simulink model "sm_wheel_loader_steer"  (R2025a)
settings: Solver=ode23t  StartTime=0.0  StopTime=70  RelTol=1e-3  AbsTol=1e-3
libraries: fl_lib x13, sm_wheel_loader_lib x6, sm_lib x3, SimscapeFluids_lib x1, nesl_utility x1
CloseFcn:
  | clear simlog_sm_wheel_loader_steering
  | clear logsout_sm_wheel_loader_steering
Description:
  | Copyright 2024-2025 The MathWorks, Inc.
settings Model: Creator=smiller  LastModifiedBy=smiller
settings SolverCC: AutoScaleAbsTol=off  AlgebraicLoopSolver=TrustRegion  MaxZcPerStep=1.0
settings DataIOCC: MaxDataPoints=10000  ReturnWorkspaceOutputs=off  SignalLoggingName=logsout_sm_wheel_loader_steer
settings DebuggingCC: UnconnectedInputMsg=warning  UnconnectedOutputMsg=warning  UnconnectedLineMsg=warning  SymbolicDimsDataTypeCodeGenerationDiagnostic=none
settings ModelReferenceCC: EnableRefExpFcnMdlSchedulingChecks=on
settings SFSimCC: CustomCodeUndefinedFunction=UseInterfaceOnly
settings RTWCC: GPUComputeCapability=3.5  DLArmComputeVersion=19.05
settings SimscapeCC: SimscapeLogType=all  SimscapeLogSimulationStatistics=on  SimscapeLogName=simlog_sm_wheel_loader_steer  SimscapeLogLimitData=off  SimscapeLogDataHistory=10000.0
settings DiagnosticsConfigSet: SimMechanicsUnconnectedFramePorts=none  SimMechanicsConflictingReferenceFrames=none
settings ExplorerConfigSet: InternalSimMechanicsExplorerSettings="<ExplorerConfiguration><canonicalview>default</canonicalview><AnimationSetting><BasePlaybackSpeed>1.0</BasePlaybackSpeed><PlaybackSpeedFactor>4.0</PlaybackSpeedFactor></AnimationSetting><TilePanel><TileInfo><Tiles Columns=\"2\" Count=\"2\" Rows=\"1\"><Column Weight=\"0.6653\"/><Column Weight=\"0.3347\"/><Row Weight=\"1\"/><Tile Height=\"1\" Width=\"1\" X=\"0\" Y=\"0\"/><Tile Height=\"1\" Width=\"1\" X=\"1\" Y=\"0\"/></Tiles></TileInfo><SceneInfo><SceneViewer><BGColor><R>1</R><G>1</G><B>1</B></BGColor><Camera><DoPerspective>off</DoPerspective><Position><X>-1.6762096275510312</X><Y>0.728440342877136993</Y><Z>1.10654866732435075</Z></Position><Center><X>0.0428012803943581543</X><Y>-0.54445752799199687</Y><Z>0.718090657281730271</Z></Center><Up><X>0.119453996973749921</X><Y>-0.138700664007791685</Y><Z>0.983103691586392436</Z></Up><ViewLimDist>1</ViewLimDist><YLim>1.24637641191482551</YLim><XLim>1.81390332452052538</XLim></Camera></SceneViewer><SceneViewer><BGColor><R>1</R><G>1</G><B>1</B></BGColor><Camera><DoPerspective>off</DoPerspective><Position><X>-0.00158637108359876988</X><Y>-0.516274428727865775</Y><Z>2.77862548640084928</Z></Position><Center><X>-0.00158637108359876988</X><Y>-0.516274428727865775</Y><Z>0.769944142090598582</Z></Center><Up><X>0</X><Y>1</Y><Z>-0</Z></Up><ViewLimDist>1</ViewLimDist><YLim>1.5781351590156556</YLim><XLim>1.14974470429161602</XLim></Camera></SceneViewer></SceneInfo></TilePanel><MechEditorPanel><Cameras/><GfxPanelCameraMap/><VideoCreator><PlaybackSpeedRatio>1.0</PlaybackSpeedRatio><FrameRate>30</FrameRate><VideoFormat>Motion JPEG AVI</VideoFormat><FrameSize>auto</FrameSize></VideoCreator></MechEditorPanel></ExplorerConfiguration>"

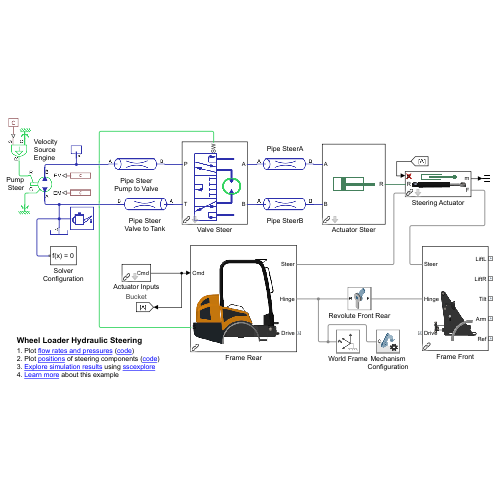
[thumbnail: Simulink's stored preview of the top-level diagram]
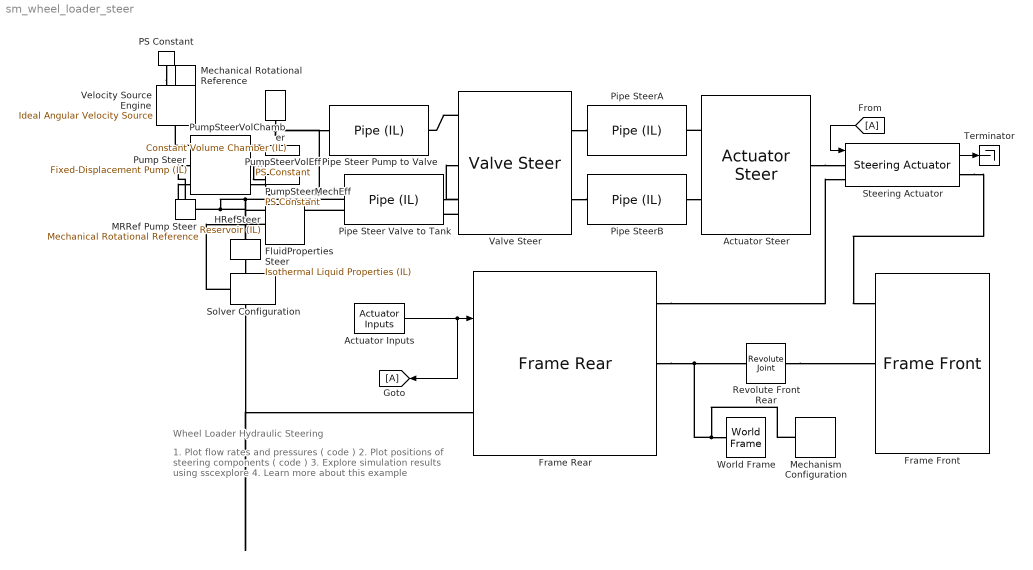
== system sm_wheel_loader_steer ==
  note: Wheel Loader Hydraulic Steering
  note: 1. Plot flow rates and pressures ( code )
      | 2. Plot positions of steering components ( code )
      | 3. Explore simulation results using sscexplore
      | 4. Learn more about this example
  Actuator Inputs : sm_wheel_loader_lib/Actuator Inputs  popup_steering=on  popup_linkage=on  popup_impl=Bucket
      settings: AttributesFormatString=%<popup_impl>
  Actuator Steer : sm_wheel_loader_lib/Wheel Loader Vehicle/Actuators/Hydraulic/Actuator Steer
  FluidProperties Steer : fl_lib/Isothermal Liquid/Utilities/Isothermal Liquid Properties (IL)  rho_L_atm=870 kg/m^3  bulk_modulus_model=foundation.enum.bulk_modulus_model.const  beta_gain=6  beta_L_atm=1.45e9 Pa  nu_atm=46 mm^2/s  p_atm=0.101325 MPa  p_min=0.1 Pa  properties_range_check=simscape.enum.assert.action.error  air_fraction=0.005  polytropic_index=1.0  rho_g_atm=1.225 kg/m^3  air_dissolution_model=simscape.enum.onoff.off  p_crit=3 MPa
  Frame Front : sm_wheel_loader_lib/Wheel Loader Vehicle/Frame Front  SystemSampleTime=-1  VariantActivationTime=update diagram  EmptyChoice=off  PassThrough=off  PassThroughVariantControl=(default)  EmptyChoiceVariantControl=(default)  AllowFlexibleInterface=on  Latency=0  AutoFrameSizeCalculation=off
  Frame Rear : sm_wheel_loader_lib/Wheel Loader Vehicle/Frame Rear  SystemSampleTime=-1  VariantActivationTime=update diagram  EmptyChoice=off  PassThrough=off  PassThroughVariantControl=(default)  EmptyChoiceVariantControl=(default)  AllowFlexibleInterface=on  Latency=0  AutoFrameSizeCalculation=off
  From : From
  Goto : Goto
  HRefSteer : fl_lib/Isothermal Liquid/Elements/Reservoir (IL)  reservoir_type=foundation.enum.constant_controlled.constant  pressure_spec=foundation.enum.pressure_spec.atmospheric  reservoir_pressure=0.101325 MPa
  MRRef Pump Steer : fl_lib/Mechanical/Rotational Elements/Mechanical Rotational Reference
  Mechanical Rotational Reference : fl_lib/Mechanical/Rotational Elements/Mechanical Rotational Reference
  Mechanism Configuration : sm_lib/Utilities/Mechanism Configuration  UniformGravity=Constant  GravityVector=[0 0 -9.80665]  GravityVectorUnits=m/s^2  LinearizationDelta=0.001  JointModeTransitionNonlinearIterations=2
  PS Constant : fl_lib/Physical Signals/Sources/PS Constant  constant=HMPST.Eng.wTarget rpm
  Pipe Steer Pump to Valve : fl_lib/Isothermal Liquid/Elements/Pipe (IL)  length=HydFcnParams.pipes.length mm  area=HydFcnParams.pipe.crossSectArea mm^2  Dh=HydFcnParams.pipes.hydraulicDiam mm  length_add=1 m  roughness=15e-6 m  Re_lam=2000  Re_tur=4000  shape_factor=64  dynamic_compressibility=simscape.enum.onoff.off  inertia=simscape.enum.onoff.off  p0=0.101325 MPa  mdot0=0 kg/s
      settings: InternalSimscapePortConfiguration="{\"Bottom\":[],\"Left\":[{\"id\":\"A\",\"label\":\"A\",\"type\":\"foundation.isothermal_liquid.isothermal_liquid\"}],\"Right\":[{\"id\":\"B\",\"label\":\"B\",\"type\":\"foundation.isothermal_liquid.isothermal_liquid\"}],\"Top\":[]}"
  Pipe Steer Valve to Tank : fl_lib/Isothermal Liquid/Elements/Pipe (IL)  length=HydFcnParams.pipes.length mm  area=HydFcnParams.pipe.crossSectArea mm^2  Dh=HydFcnParams.pipes.hydraulicDiam mm  length_add=1 m  roughness=15e-6 m  Re_lam=2000  Re_tur=4000  shape_factor=64  dynamic_compressibility=simscape.enum.onoff.off  inertia=simscape.enum.onoff.off  p0=0.101325 MPa  mdot0=0 kg/s
      settings: InternalSimscapePortConfiguration="{\"Bottom\":[],\"Left\":[{\"id\":\"A\",\"label\":\"A\",\"type\":\"foundation.isothermal_liquid.isothermal_liquid\"}],\"Right\":[{\"id\":\"B\",\"label\":\"B\",\"type\":\"foundation.isothermal_liquid.isothermal_liquid\"}],\"Top\":[]}"
  Pipe SteerA : fl_lib/Isothermal Liquid/Elements/Pipe (IL)  length=HydFcnParams.pipes.length mm  area=HydFcnParams.pipe.crossSectArea mm^2  Dh=HydFcnParams.pipes.hydraulicDiam mm  length_add=1 m  roughness=15e-6 m  Re_lam=2000  Re_tur=4000  shape_factor=64  dynamic_compressibility=simscape.enum.onoff.off  inertia=simscape.enum.onoff.off  p0=0.101325 MPa  mdot0=0 kg/s
      settings: InternalSimscapePortConfiguration="{\"Bottom\":[],\"Left\":[{\"id\":\"A\",\"label\":\"A\",\"type\":\"foundation.isothermal_liquid.isothermal_liquid\"}],\"Right\":[{\"id\":\"B\",\"label\":\"B\",\"type\":\"foundation.isothermal_liquid.isothermal_liquid\"}],\"Top\":[]}"
  Pipe SteerB : fl_lib/Isothermal Liquid/Elements/Pipe (IL)  length=HydFcnParams.pipes.length mm  area=HydFcnParams.pipe.crossSectArea mm^2  Dh=HydFcnParams.pipes.hydraulicDiam mm  length_add=1 m  roughness=15e-6 m  Re_lam=2000  Re_tur=4000  shape_factor=64  dynamic_compressibility=simscape.enum.onoff.off  inertia=simscape.enum.onoff.off  p0=0.101325 MPa  mdot0=0 kg/s
      settings: InternalSimscapePortConfiguration="{\"Bottom\":[],\"Left\":[{\"id\":\"A\",\"label\":\"A\",\"type\":\"foundation.isothermal_liquid.isothermal_liquid\"}],\"Right\":[{\"id\":\"B\",\"label\":\"B\",\"type\":\"foundation.isothermal_liquid.isothermal_liquid\"}],\"Top\":[]}"
  Pump Steer : SimscapeFluids_lib/Isothermal Liquid/Pumps & Motors/Fixed-Displacement Pump (IL)  leakage_friction_spec=fluids.isothermal_liquid.pumps_motors.enum.pump_motor_loss_spec.input_efficiency  displacement=HydFcnParams.steerPump.displacement cm^3/rev  omega_nominal=HydFcnParams.pump.nomSpeed rpm  p_nominal=HydFcnParams.pump.nomPrGain bar  vol_eff_nominal=HydFcnParams.pump.volEff  mech_eff_nominal=HydFcnParams.pump.mechEff  no_load_torque=0 N*m  p_diff_eff_TLU=[.1, 1, 2] MPa  omega_eff_TLU=[250, 500, 1000, 2000, 3000, 4000] rpm  vol_eff_TLU=[.816, .908, .954, .977, .981, .984; .325, .663, .831, .916, .925, .946; .137, .568, .78, .892, .893, .91]  mech_eff_TLU=[.996, .996, .996, .996, .996, .996; .988, .989, .989, .989, .989, .99; .981, .981, .982, .982, .983, .984]  p_diff_loss_TLU=[.1, 1, 2] MPa  omega_loss_TLU=[250, 500, 1000, 2000, 3000, 4000] rpm  vol_loss_TLU=1e-3 * [.023, .023, .023, .023, .0285, .032; .0844, .0842, .0845, .084, .1125, .108; .1079, .108, .11, .108, .1605, .18] m^3/s  mech_loss_TLU=[.002, .002, .002, .002, .002, .002; .0607, .0556, .0556, .0556, .0556, .0505; .1937, .1937, .1833, .1833, .1729, .1626] N*m  vol_eff_min=1e-3  vol_eff_max=1  mech_eff_min=1e-3  mech_eff_max=1  pressure_threshold=1e-3 MPa  omega_threshold=100 rpm  supplied_range_check=simscape.enum.assert.action.none  pump_mode_check=simscape.enum.assert.action.none  pressure_check=simscape.enum.assert.action.none  p_min_valid=0.101325 MPa
      settings: InternalSimscapePortConfiguration="{\"Bottom\":[{\"id\":\"A\",\"label\":\"A\",\"type\":\"foundation.isothermal_liquid.isothermal_liquid\"}],\"Left\":[{\"id\":\"EV\",\"label\":\"EV\",\"type\":\"input\"},{\"id\":\"EM\",\"label\":\"EM\",\"type\":\"input\"}],\"Right\":[{\"id\":\"R\",\"label\":\"R\",\"type\":\"foundation.mechanical.rotational.rotational\"},{\"id\":\"C\",\"label\":\"C\",\"type\":\"foundation.mechanical.rotational.rotational\"}],\"Top\":[{\"id\":\"B\",\"label\":\"B\",\"type\":\"foundation.isothermal_liquid.isothermal_liquid\"}]}"
  PumpSteerMechEff : fl_lib/Physical Signals/Sources/PS Constant  constant=HydFcnParams.steerPump.mechEff
  PumpSteerVolChamber : fl_lib/Isothermal Liquid/Elements/Constant Volume Chamber (IL)  volume=HydFcnParams.steerPump.chamberVol mm^3  p_I_specify=off  p_I_priority=High  p_I=0.101325 MPa  p_I_nominal_specify=off  p_I_nominal_value=1  p_I_nominal_unit=MPa
      settings: InternalSimscapePortConfiguration="{\"Bottom\":[],\"Left\":[{\"id\":\"A\",\"label\":\"A\",\"type\":\"foundation.isothermal_liquid.isothermal_liquid\"}],\"Right\":[],\"Top\":[]}"
  PumpSteerVolEff : fl_lib/Physical Signals/Sources/PS Constant  constant=HydFcnParams.steerPump.volEff
  Revolute Front Rear : sm_lib/Joints/Revolute Joint  JointMode=Normal  CompositeWrenchDir=FollowerOnBase  CompositeWrenchFrame=BaseFrame  SenseConstraintForce=off  SenseConstraintTorque=off  SenseTotalForce=off  SenseTotalTorque=off  PositionTargetSpecify=off  PositionTargetPriority=High  PositionTargetValue=0  PositionTargetValueUnits=deg  VelocityTargetSpecify=off  VelocityTargetPriority=High  VelocityTargetValue=0  VelocityTargetValueUnits=deg/s  EquilibriumPosition=0  EquilibriumPositionUnits=deg  SpringStiffness=0  SpringStiffnessUnits=N*m/deg  DampingCoefficient=0  DampingCoefficientUnits=N*m/(rad/s)  LowerLimitSpecify=off  LowerLimitBound=-90  LowerLimitBoundUnits=deg  LowerLimitStiffness=1e4  LowerLimitStiffnessUnits=N*m/deg  LowerLimitDamping=10  LowerLimitDampingUnits=N*m/(deg/s)  LowerLimitTransitionRegionWidth=0.1  LowerLimitTransitionRegionWidthUnits=deg  UpperLimitSpecify=off  UpperLimitBound=90  UpperLimitBoundUnits=deg  UpperLimitStiffness=1e4  UpperLimitStiffnessUnits=N*m/deg  UpperLimitDamping=10  UpperLimitDampingUnits=N*m/(deg/s)  UpperLimitTransitionRegionWidth=0.1  UpperLimitTransitionRegionWidthUnits=deg  TorqueActuationMode=NoTorque  MotionActuationMode=ComputedMotion  SensePosition=off  SenseVelocity=off  SenseAcceleration=off  SenseTorqueForce=off  SenseLowerLimitTorqueForce=off  SenseUpperLimitTorqueForce=off
  Solver Configuration : nesl_utility/Solver Configuration  PhysicalDomain=network_engine_domain  SubClassName=solver  LeftPortType=input  RightPortType=generic  Tones=[]  Harmonics=[]  SimulateNoise=off  Profile=off  UseLocalSampling=off  EnableSwitchedLinearOptims=on  FrequencyDomain=off  UseCCode=off  RelTol=0.001  AbsTol=1e-06  MinStep=1e-09  ToWorkspace=off  RevertToSquareIcSolve=off  NumHomotopyIterations=100  PhasorMode=off  PhasorModeNumHarmonics=1  ConsistencySolver=NEWTON_XTOL_AFTER_FTOL  IndexReductionMethod=DerivativeReplacement  DoDC=off  ResidualTolerance=1e-09  ConsistencyTolSource=GLOBAL  ConsistencyAbsTol=0.001  ConsistencyRelTol=0.001  ConsistencyTolFactor=0.001  UseLocalSolver=off  LocalSolverChoice=NE_BACKWARD_EULER_ADVANCER  ResolveIndetEquations=on  FunctionEvalNumThread=1  LocalSolverSampleTime=0.001  DoFixedCost=off  MaxNonlinIter=3  MaxModeIter=2  ComputeImpulses=off  ImpulseIterations=2  LinearAlgebra=auto  LinearAlgebraNumThread=0  EquationFormulation=NE_TIME_EF  DelaysMemoryBudget=1024  AutomaticFiltering=on  FilteringTimeConstant=0.001  PartitionStorageMethod=AS_NEEDED  PartitionMemoryBudget=1024  PartitionMethod=ROBUST  MultibodyUseLocalSolver=off  MultibodyLocalSolverChoice=ODE1  MultibodyLocalSolverSampleTime=0.001
  Steering Actuator : sm_wheel_loader_lib/Wheel Loader Vehicle/Steering Actuator  popup_actuator_model=Shaft
  Terminator : Terminator
  Valve Steer : sm_wheel_loader_lib/Wheel Loader Vehicle/Actuators/Hydraulic/Valve Steer
  Velocity Source Engine : fl_lib/Mechanical/Mechanical Sources/Ideal Angular Velocity Source
  World Frame : sm_lib/Frames and Transforms/World Frame
  wires:
  From/1 -> Steering Actuator/1
  Actuator Inputs/1 -> Frame Rear/1, Goto/1
  Steering Actuator/1 -> Terminator/1
  connections:
  PumpSteerVolChamber/LConn1 -- Pump Steer/LConn3 -- Pipe Steer Pump to Valve/LConn1
  Pump Steer/RConn3 -- Pipe Steer Valve to Tank/RConn1 -- Solver Configuration/RConn1 -- HRefSteer/LConn1 -- FluidProperties Steer/RConn1
  Valve Steer/LConn3 -- Frame Rear/LConn1
  Pipe Steer Valve to Tank/LConn1 -- Valve Steer/LConn2
  Valve Steer/RConn2 -- Pipe SteerB/LConn1
  Actuator Steer/LConn1 -- Pipe SteerA/RConn1
  Pump Steer/LConn2 -- PumpSteerMechEff/RConn1
  MRRef Pump Steer/LConn1 -- Pump Steer/RConn2
  Actuator Steer/RConn1 -- Steering Actuator/LConn1
  PumpSteerVolEff/RConn1 -- Pump Steer/LConn1
  Valve Steer/RConn1 -- Pipe SteerA/LConn1
  Valve Steer/LConn1 -- Pipe Steer Pump to Valve/RConn1
  Pipe SteerB/RConn1 -- Actuator Steer/LConn2
  PS Constant/RConn1 -- Velocity Source Engine/RConn1
  Pump Steer/RConn1 -- Velocity Source Engine/LConn1
  Velocity Source Engine/RConn2 -- Mechanical Rotational Reference/LConn1
  Mechanism Configuration/RConn1 -- Frame Rear/RConn2 -- Revolute Front Rear/LConn1 -- World Frame/RConn1
  Revolute Front Rear/RConn1 -- Frame Front/LConn2
  Steering Actuator/RConn1 -- Frame Front/LConn1
  Frame Rear/RConn1 -- Steering Actuator/LConn2
